simulink model "Lab_2_2_2_observer_design"  (R2024b)
settings: Solver=VariableStepAuto  StartTime=0.0  StopTime=10  RelTol=1e-3
undefined symbols (not defined in the file): Gamma, Gamma_o, H, H_o, J, J_o, K, Nr, Phi, Phi_o, Ts
libraries: simulink_extras x2
settings Model: Creator=vahid  LastModifiedBy=vahid

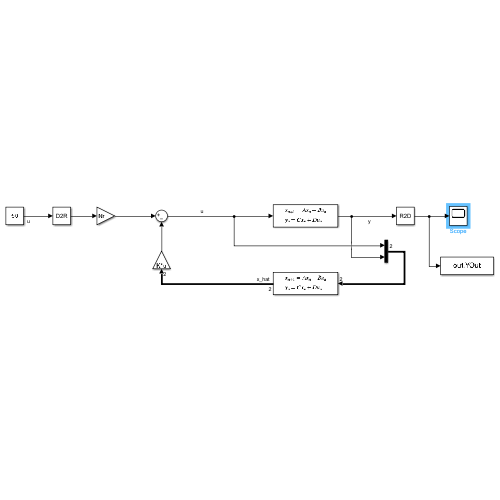
[thumbnail: Simulink's stored preview of the top-level diagram]
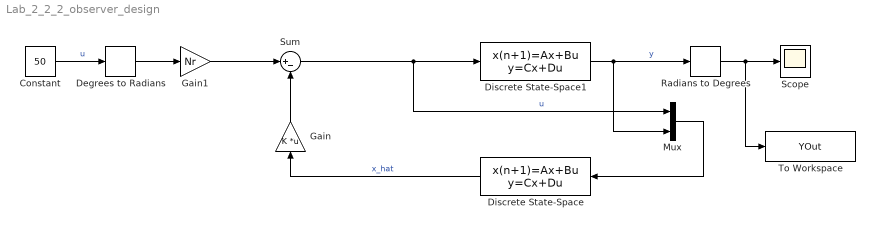
== system Lab_2_2_2_observer_design ==
  Constant : Constant  Value=50
  Degrees to Radians : simulink_extras/Transformations/Degrees to Radians
  Discrete State-Space : DiscreteStateSpace  A=Phi_o  B=Gamma_o  C=H_o  D=J_o  SampleTime=Ts
  Discrete State-Space1 : DiscreteStateSpace  A=Phi  B=Gamma  C=H  D=J  SampleTime=Ts
  Gain : Gain  Gain=K  Multiplication=Matrix(K*u)
  Gain1 : Gain  Gain=Nr
  Mux : Mux  Inputs=2
  Radians to Degrees : simulink_extras/Transformations/Radians to Degrees
  Scope : Scope
  Sum : Sum  Inputs=|+-
  To Workspace : ToWorkspace  VariableName=YOut  SaveFormat=Timeseries  SampleTime=-1
  wires:
  Sum/1 -> Mux/1, Discrete State-Space1/1  "u"
  Discrete State-Space1/1 -> Mux/2, Radians to Degrees/1  "y"
  Mux/1 -> Discrete State-Space/1
  Discrete State-Space/1 -> Gain/1  "x_hat"
  Constant/1 -> Degrees to Radians/1  "u"
  Gain/1 -> Sum/2
  Gain1/1 -> Sum/1
  Degrees to Radians/1 -> Gain1/1
  Radians to Degrees/1 -> To Workspace/1, Scope/1
